simulink model "dab_openloop_fixed_step_interpolation"  (R2024b)
settings: Solver=ode1be  StartTime=0.0  StopTime=T_stop  FixedStep=TFIX  MaxStep=Tsolver  RelTol=1e-05
values from neighbouring files (symbols this model uses):
  Ci = 30e-6*s_f    (= 7.5e-05)    [init.m]
  Co = 44e-6*s_f    (= 0.00011)    [init.m]
  D1_OL = 0.985714    [init.m]
  D2_OL = 1    [init.m]
  D3_OL = 0.045188    [init.m]
  ESR_Ci = 2e-3    (= 0.002)    [init.m]
  ESR_Co = 2e-3    (= 0.002)    [init.m]
  f_sw = 20e3    (= 20000)    [init.m]
  Li = 10e-6*s_f    (= 2.5e-05)    [init.m]
  Lo = 10e-6*s_f    (= 2.5e-05)    [init.m]
  Rd_diode = 8e-3    (= 0.008)    [init.m]
  Ri = 100e-3    (= 0.1)    [init.m]
  Ro = 100e-3    (= 0.1)    [init.m]
  Ron = 3.5e-3    (= 0.0035)    [init.m]
  Rs_snub = 1e5    (= 100000)    [init.m]
  tdead = 200e-9    (= 2e-07)    [init.m]
  TFIX = 20e-9    (= 2e-08)    [init.m]    (also in run_fixed_step_100ns.m = 1e-07; run_fixed_step_20ns.m; run_fixed_step_interpolation_100ns.m = 1e-07; run_fixed_step_interpolation_20ns.m)
  Tp = 1/f_sw    (= 5e-05)    [init.m]
  TR_fn = f_sw    (= 20000)    [init.m]
  TR_Lm = 1    [init.m]
  TR_Pn = 30e3    (= 30000)    [init.m]
  TR_Rm = 1e6    (= 1000000)    [init.m]
  V_cap_init = Vi - Ri*IL0_i    (= 797.500025)    [init.m]
  V_out_init = Vo + Ro*I_OP    (= 454.4444)    [init.m]
  Vf_diode = 3.0    (= 3)    [init.m]
  Vi = 800    [init.m]
  Vo = V_BAT    (= 450)    [init.m]
libraries: spsSeriesRLCBranchLib x16, spsControlledVoltageSourceLib x6, spsCurrentMeasurementLib x3, spsControlledCurrentSourceLib x2, spsGroundLib x2, spsVoltageMeasurementLib x2, spsLinearTransformerLib x1, sps_lib x1
settings Model: Creator=amina  LastModifiedBy=amina
settings SolverCC: MaxConsecutiveMinStep=100
settings DataIOCC: SaveOutput=off  SignalLogging=off  DSMLogging=off  SaveTime=off  ReturnWorkspaceOutputsName=out_analytic

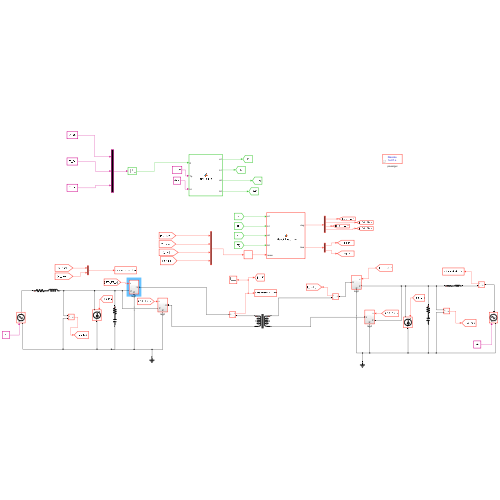
[thumbnail: Simulink's stored preview of the top-level diagram]
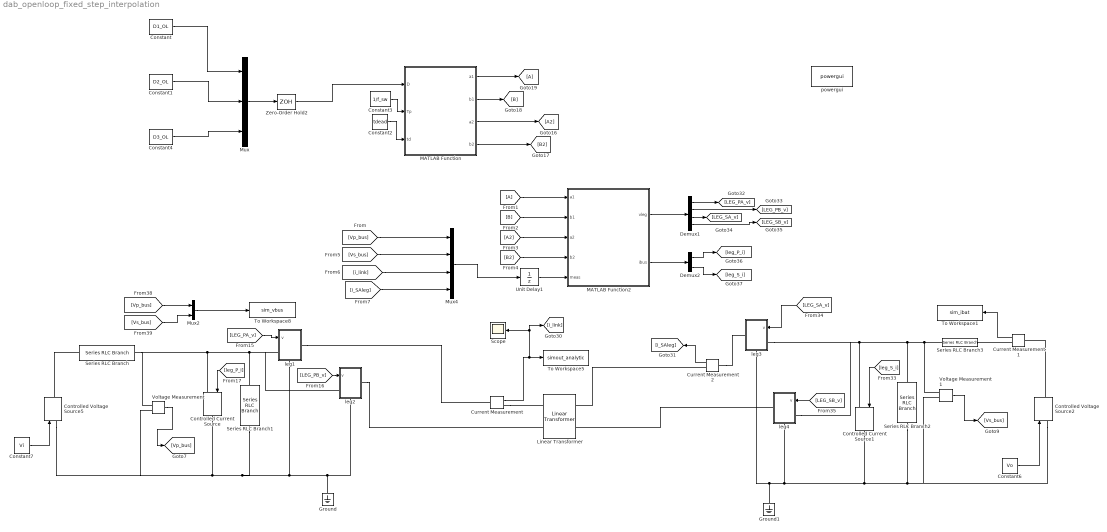
== system dab_openloop_fixed_step_interpolation ==
  Constant : Constant  Value=D1_OL
  Constant1 : Constant  Value=D2_OL
  Constant2 : Constant  Value=tdead
  Constant3 : Constant  Value=1/f_sw
  Constant4 : Constant  Value=D3_OL
  Constant6 : Constant  Value=Vo
  Constant7 : Constant  Value=Vi
  Controlled Current Source : spsControlledCurrentSourceLib/Controlled Current Source  Initialize=off  Source_Type=AC  Amplitude=0  Phase=0  Frequency=0  Measurements=None
  Controlled Current Source1 : spsControlledCurrentSourceLib/Controlled Current Source  Initialize=off  Source_Type=AC  Amplitude=0  Phase=0  Frequency=0  Measurements=None
  Controlled Voltage Source2 : spsControlledVoltageSourceLib/Controlled Voltage Source  Initialize=on  Source_Type=DC  Amplitude=Vo  Phase=0  Frequency=0  Measurements=None
  Controlled Voltage Source5 : spsControlledVoltageSourceLib/Controlled Voltage Source  Initialize=on  Source_Type=DC  Amplitude=Vi  Phase=0  Frequency=0  Measurements=None
  Current Measurement : spsCurrentMeasurementLib/Current Measurement  PhasorSimulation=off  OutputType=Complex  PSBequivalent=0
  Current Measurement1 : spsCurrentMeasurementLib/Current Measurement  PhasorSimulation=off  OutputType=Complex  PSBequivalent=0
  Current Measurement2 : spsCurrentMeasurementLib/Current Measurement  PhasorSimulation=off  OutputType=Complex  PSBequivalent=0
  Demux1 : Demux
  Demux2 : Demux  Outputs=2
  From1 : From
  Goto19 : Goto
  Ground : spsGroundLib/Ground  LConnTagsString=a
  Ground1 : spsGroundLib/Ground  LConnTagsString=a
  Linear Transformer : spsLinearTransformerLib/Linear Transformer  UNITS=SI  NominalPower=[TR_Pn TR_fn]  winding1=TR_W1  winding2=TR_W2  ThreeWindings=off  winding3=[3.15e+05 0.7938 0.084225]  RmLm=[TR_Rm TR_Lm]  Measurements=None  DataType=on
  MATLAB Function : MATLAB Function  TreatAsAtomicUnit=on
  MATLAB Function2 : MATLAB Function  TreatAsAtomicUnit=on
  Mux : Mux  Inputs=3
  Mux2 : Mux  Inputs=2
  Mux4 : Mux
  Scope : Scope
  Series RLC Branch : spsSeriesRLCBranchLib/Series RLC Branch  LConnTagsString=__new0  RConnTagsString=__new0  BranchType=RL  Resistance=Ri  Inductance=Li  SetiL0=on  InitialCurrent=IL0_i  Capacitance=1e-6  Setx0=off  InitialVoltage=0  Measurements=None
  Series RLC Branch1 : spsSeriesRLCBranchLib/Series RLC Branch  LConnTagsString=__new0  RConnTagsString=__new0  BranchType=RC  Resistance=ESR_Ci  Inductance=1e-3  SetiL0=off  InitialCurrent=0  Capacitance=Ci  Setx0=on  InitialVoltage=V_cap_init  Measurements=None
  Series RLC Branch2 : spsSeriesRLCBranchLib/Series RLC Branch  LConnTagsString=__new0  RConnTagsString=__new0  BranchType=RC  Resistance=ESR_Co  Inductance=1e-3  SetiL0=off  InitialCurrent=0  Capacitance=Co  Setx0=on  InitialVoltage=V_out_init  Measurements=None
  Series RLC Branch3 : spsSeriesRLCBranchLib/Series RLC Branch  LConnTagsString=__new0  RConnTagsString=__new0  BranchType=RL  Resistance=Ro  Inductance=Lo  SetiL0=on  InitialCurrent=IL0_o  Capacitance=1e-6  Setx0=off  InitialVoltage=0  Measurements=None
  To Workspace1 : ToWorkspace  VariableName=sim_ibat  SaveFormat=Timeseries  SampleTime=-1
  To Workspace5 : ToWorkspace  VariableName=simout_analytic  SaveFormat=Timeseries  SampleTime=-1
  To Workspace8 : ToWorkspace  VariableName=sim_vbus  SaveFormat=Timeseries  SampleTime=-1
  Unit Delay1 : UnitDelay  InitialCondition=[V_cap_init; V_out_init; 0; 0]  SampleTime=TFIX  HasFrameUpgradeWarning=on
  Voltage Measurement : spsVoltageMeasurementLib/Voltage Measurement  PhasorSimulation=off  OutputType=Complex  PSBequivalent=0
  Voltage Measurement1 : spsVoltageMeasurementLib/Voltage Measurement  PhasorSimulation=off  OutputType=Complex  PSBequivalent=0
  Zero-Order Hold2 : ZeroOrderHold  SampleTime=1/f_sw
  leg1 : Subsystem
      settings: PortSchema="{\"entries\":[{\"content\":{\"sides\":[{\"content\":{\"connectorIds\":[\"In1\",\"LConn1\"]},\"type\":\"ConnectorPlacement.EquallySpacedRectSide\",\"uuid\":\"81142e03-bbe8-4655-b0fc-f40d7cb28308\"},{\"content\":{\"connectorIds\":[\"RConn1\"],\"side\":\"RIGHT\"},\"type\":\"ConnectorPlacement.EquallySpacedRectSide\",\"uuid\":\"8b0fa82a-ef23-4d29-b267-a4b058b7878b\"},{\"content\":{\"side\":\"TOP\"},\"type\":\"ConnectorPlacement.EquallySpacedRectSide\",\"uuid\":\"6ef32b7f-a709-442f-b038-19cc6fffc8df\"},{\"content\":{\"connectorIds\":[\"RConn2\"],\"side\":\"BOTTOM\"},\"type\":\"ConnectorPlacement.EquallySpacedRectSide\",\"uuid\":\"acaab421-7729-4a20-97ce-5be0a5a8c4d3\"}]},\"type\":\"ConnectorPlacement.EquallySpacedConnector\",\"uuid\":\"423ad79b-2f01-454b-b2f3-d9f36115acf4\"}],\"packageUris\":[\"http://schema.mathworks.com/mf0/Connector/R2020b\"],\"version\":\"1.0\"}"
  leg2 : Subsystem
      settings: PortSchema="{\"entries\":[{\"content\":{\"sides\":[{\"content\":{\"connectorIds\":[\"In1\",\"LConn1\"]},\"type\":\"ConnectorPlacement.EquallySpacedRectSide\",\"uuid\":\"81142e03-bbe8-4655-b0fc-f40d7cb28308\"},{\"content\":{\"connectorIds\":[\"RConn1\"],\"side\":\"RIGHT\"},\"type\":\"ConnectorPlacement.EquallySpacedRectSide\",\"uuid\":\"8b0fa82a-ef23-4d29-b267-a4b058b7878b\"},{\"content\":{\"side\":\"TOP\"},\"type\":\"ConnectorPlacement.EquallySpacedRectSide\",\"uuid\":\"6ef32b7f-a709-442f-b038-19cc6fffc8df\"},{\"content\":{\"connectorIds\":[\"RConn2\"],\"side\":\"BOTTOM\"},\"type\":\"ConnectorPlacement.EquallySpacedRectSide\",\"uuid\":\"acaab421-7729-4a20-97ce-5be0a5a8c4d3\"}]},\"type\":\"ConnectorPlacement.EquallySpacedConnector\",\"uuid\":\"423ad79b-2f01-454b-b2f3-d9f36115acf4\"}],\"packageUris\":[\"http://schema.mathworks.com/mf0/Connector/R2020b\"],\"version\":\"1.0\"}"
  leg3 : Subsystem
      settings: PortSchema="{\"entries\":[{\"content\":{\"sides\":[{\"content\":{\"connectorIds\":[\"In1\",\"LConn1\"]},\"type\":\"ConnectorPlacement.EquallySpacedRectSide\",\"uuid\":\"81142e03-bbe8-4655-b0fc-f40d7cb28308\"},{\"content\":{\"connectorIds\":[\"RConn1\"],\"side\":\"RIGHT\"},\"type\":\"ConnectorPlacement.EquallySpacedRectSide\",\"uuid\":\"8b0fa82a-ef23-4d29-b267-a4b058b7878b\"},{\"content\":{\"side\":\"TOP\"},\"type\":\"ConnectorPlacement.EquallySpacedRectSide\",\"uuid\":\"6ef32b7f-a709-442f-b038-19cc6fffc8df\"},{\"content\":{\"connectorIds\":[\"RConn2\"],\"side\":\"BOTTOM\"},\"type\":\"ConnectorPlacement.EquallySpacedRectSide\",\"uuid\":\"acaab421-7729-4a20-97ce-5be0a5a8c4d3\"}]},\"type\":\"ConnectorPlacement.EquallySpacedConnector\",\"uuid\":\"423ad79b-2f01-454b-b2f3-d9f36115acf4\"}],\"packageUris\":[\"http://schema.mathworks.com/mf0/Connector/R2020b\"],\"version\":\"1.0\"}"
  leg4 : Subsystem
      settings: PortSchema="{\"entries\":[{\"content\":{\"sides\":[{\"content\":{\"connectorIds\":[\"In1\",\"LConn1\"]},\"type\":\"ConnectorPlacement.EquallySpacedRectSide\",\"uuid\":\"81142e03-bbe8-4655-b0fc-f40d7cb28308\"},{\"content\":{\"connectorIds\":[\"RConn1\"],\"side\":\"RIGHT\"},\"type\":\"ConnectorPlacement.EquallySpacedRectSide\",\"uuid\":\"8b0fa82a-ef23-4d29-b267-a4b058b7878b\"},{\"content\":{\"side\":\"TOP\"},\"type\":\"ConnectorPlacement.EquallySpacedRectSide\",\"uuid\":\"6ef32b7f-a709-442f-b038-19cc6fffc8df\"},{\"content\":{\"connectorIds\":[\"RConn2\"],\"side\":\"BOTTOM\"},\"type\":\"ConnectorPlacement.EquallySpacedRectSide\",\"uuid\":\"acaab421-7729-4a20-97ce-5be0a5a8c4d3\"}]},\"type\":\"ConnectorPlacement.EquallySpacedConnector\",\"uuid\":\"423ad79b-2f01-454b-b2f3-d9f36115acf4\"}],\"packageUris\":[\"http://schema.mathworks.com/mf0/Connector/R2020b\"],\"version\":\"1.0\"}"
  powergui : sps_lib/powergui  Priority=1  SimulationMode=Discrete  SampleTime=TFIX  frequency=60  Iterations=50  frequencyindice=0  Pbase=100e6  ErrMax=1e-4  UnitsV=kV  UnitsW=MW  buscounter=0  FunctionMessages=off  echomessages=off  EnableUseOfTLC=off  CurrentSourceSwitches=off  DisableSnubberDevices=off  DisableRonSwitches=off  DisableVfSwitches=off  DisplayEquations=off  AutomaticDiscreteSolvers=off  SolverType=Tustin  Interpol=off  ExternalGateDelay=off  methode=off  Ts=100  x0status=blocks  SPID=on  SwTol=0  HookPort=off  NonlinearTolerance=1e-4  nMaxIteration=100  ContinueOnMaxIteration=off  RestoreLinks=warning  ResistiveCurrentMeasurement=off  Frange=[0:2:500]  Ylog=off  Xlog=on  ShowGrid=off  save=off  variable=ZData  structure=0  ZoomFFT=off  StartTime=0.0  cycles=1  DisplayStyle=1  fundamental=60  FreqAxis=off  MaxFrequency=1000  frequencyindicesteady=1  RmsSteady=1  display=off
  wires:
  Constant6/1 -> Controlled Voltage Source2/1
  Constant7/1 -> Controlled Voltage Source5/1
  Current Measurement/1 -> Scope/1, [i_link], To Workspace5/1
  Voltage Measurement/1 -> [Vp_bus]
  Voltage Measurement1/1 -> [Vs_bus]
  [Vs_bus] -> Mux2/2
  Mux2/1 -> To Workspace8/1
  [Vp_bus] -> Mux2/1
  From1/1 -> MATLAB Function2/1(a1)
  [B] -> MATLAB Function2/2(b1)
  [A2] -> MATLAB Function2/3(a2)
  [B2] -> MATLAB Function2/4(b2)
  Current Measurement2/1 -> [i_SAleg]
  [Vp_bus] -> Mux4/1
  [Vs_bus] -> Mux4/2
  [i_link] -> Mux4/3
  [i_SAleg] -> Mux4/4
  Mux4/1 -> Unit Delay1/1
  Unit Delay1/1 -> MATLAB Function2/5(meas)
  MATLAB Function2/2(ibus) -> Demux2/1
  MATLAB Function2/1(vleg) -> Demux1/1
  Demux1/1 -> [LEG_PA_v]
  Demux1/3 -> [LEG_SA_v]
  Demux1/2 -> [LEG_PB_v]
  Demux1/4 -> [LEG_SB_v]
  Demux2/1 -> [leg_P_i]
  Demux2/2 -> [leg_S_i]
  [LEG_PA_v] -> leg1/1(v)
  [LEG_PB_v] -> leg2/1(v)
  [leg_P_i] -> Controlled Current Source/1
  [leg_S_i] -> Controlled Current Source1/1
  [LEG_SA_v] -> leg3/1(v)
  [LEG_SB_v] -> leg4/1(v)
  Mux/1 -> Zero-Order Hold2/1
  Constant/1 -> Mux/1
  Constant1/1 -> Mux/2
  Constant3/1 -> MATLAB Function/2(Tp)
  MATLAB Function/4(b2) -> [B2]
  MATLAB Function/3(a2) -> [A2]
  MATLAB Function/1(a1) -> Goto19/1
  MATLAB Function/2(b1) -> [B]
  Constant2/1 -> MATLAB Function/3(td)
  Constant4/1 -> Mux/3
  Zero-Order Hold2/1 -> MATLAB Function/1(D)
  Current Measurement1/1 -> To Workspace1/1
  connections:
  leg1/RConn1 -- Current Measurement/LConn1
  Voltage Measurement/LConn1 -- Series RLC Branch/RConn1 -- Controlled Current Source/LConn1 -- leg2/LConn1 -- leg1/LConn1 -- Series RLC Branch1/LConn1
  leg1/RConn2 -- Controlled Current Source/RConn1 -- Voltage Measurement/LConn2 -- Controlled Voltage Source5/LConn1 -- Series RLC Branch1/RConn1 -- leg2/RConn2 -- Ground/LConn1
  leg2/RConn1 -- Linear Transformer/LConn2
  Voltage Measurement1/LConn1 -- leg3/LConn1 -- leg4/LConn1 -- Controlled Current Source1/LConn1 -- Series RLC Branch2/LConn1 -- Series RLC Branch3/LConn1
  Voltage Measurement1/LConn2 -- Controlled Voltage Source2/LConn1 -- Series RLC Branch2/RConn1 -- Controlled Current Source1/RConn1 -- leg4/RConn2 -- leg3/RConn2 -- Ground1/LConn1
  leg4/RConn1 -- Linear Transformer/RConn2
  Current Measurement2/RConn1 -- Linear Transformer/RConn1
  Current Measurement/RConn1 -- Linear Transformer/LConn1
  Current Measurement1/RConn1 -- Series RLC Branch3/RConn1
  Controlled Voltage Source2/RConn1 -- Current Measurement1/LConn1
  Controlled Voltage Source5/RConn1 -- Series RLC Branch/LConn1
  Current Measurement2/LConn1 -- leg3/RConn1

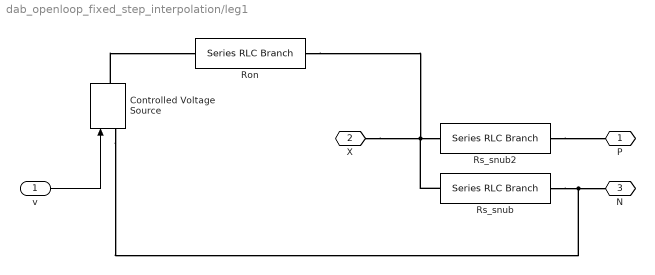
== system dab_openloop_fixed_step_interpolation/leg1 ==
  v : Inport
  Controlled Voltage Source : spsControlledVoltageSourceLib/Controlled Voltage Source  Initialize=off  Source_Type=AC  Amplitude=0  Phase=0  Frequency=0  Measurements=None
  Ron : spsSeriesRLCBranchLib/Series RLC Branch  LConnTagsString=__new0  RConnTagsString=__new0  BranchType=R  Resistance=Ron  Inductance=Li  SetiL0=on  InitialCurrent=IL0_i  Capacitance=1e-6  Setx0=off  InitialVoltage=0  Measurements=None
  Rs_snub : spsSeriesRLCBranchLib/Series RLC Branch  LConnTagsString=__new0  RConnTagsString=__new0  BranchType=R  Resistance=Rs_snub  Inductance=Li  SetiL0=on  InitialCurrent=IL0_i  Capacitance=1e-6  Setx0=off  InitialVoltage=0  Measurements=None
  Rs_snub2 : spsSeriesRLCBranchLib/Series RLC Branch  LConnTagsString=__new0  RConnTagsString=__new0  BranchType=R  Resistance=Rs_snub  Inductance=Li  SetiL0=on  InitialCurrent=IL0_i  Capacitance=1e-6  Setx0=off  InitialVoltage=0  Measurements=None
  " P" : PMIOPort  Side=Left
  X : PMIOPort  Port=2  Side=Right
  N : PMIOPort  Port=3  Side=Right
  wires:
  v/1 -> Controlled Voltage Source/1
  connections:
  Rs_snub2/RConn1 -- " P"/RConn1
  Rs_snub/LConn1 -- Rs_snub2/LConn1 -- X/RConn1 -- Ron/RConn1
  Controlled Voltage Source/LConn1 -- Rs_snub/RConn1 -- N/RConn1
  Controlled Voltage Source/RConn1 -- Ron/LConn1

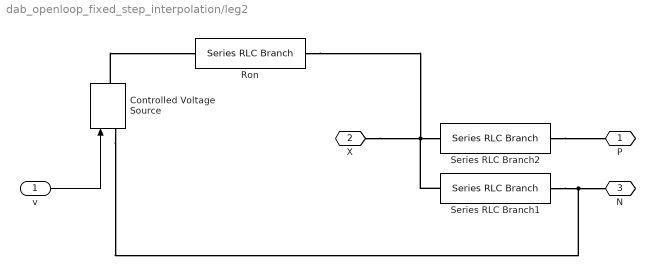
== system dab_openloop_fixed_step_interpolation/leg2 ==
  v : Inport
  Controlled Voltage Source : spsControlledVoltageSourceLib/Controlled Voltage Source  Initialize=off  Source_Type=AC  Amplitude=0  Phase=0  Frequency=0  Measurements=None
  Ron : spsSeriesRLCBranchLib/Series RLC Branch  LConnTagsString=__new0  RConnTagsString=__new0  BranchType=R  Resistance=Ron  Inductance=Li  SetiL0=on  InitialCurrent=IL0_i  Capacitance=1e-6  Setx0=off  InitialVoltage=0  Measurements=None
  Series RLC Branch1 : spsSeriesRLCBranchLib/Series RLC Branch  LConnTagsString=__new0  RConnTagsString=__new0  BranchType=R  Resistance=Rs_snub  Inductance=Li  SetiL0=on  InitialCurrent=IL0_i  Capacitance=1e-6  Setx0=off  InitialVoltage=0  Measurements=None
  Series RLC Branch2 : spsSeriesRLCBranchLib/Series RLC Branch  LConnTagsString=__new0  RConnTagsString=__new0  BranchType=R  Resistance=Rs_snub  Inductance=Li  SetiL0=on  InitialCurrent=IL0_i  Capacitance=1e-6  Setx0=off  InitialVoltage=0  Measurements=None
  " P" : PMIOPort  Side=Left
  X : PMIOPort  Port=2  Side=Right
  N : PMIOPort  Port=3  Side=Right
  wires:
  v/1 -> Controlled Voltage Source/1
  connections:
  Series RLC Branch2/RConn1 -- " P"/RConn1
  Series RLC Branch1/LConn1 -- Series RLC Branch2/LConn1 -- X/RConn1 -- Ron/RConn1
  Controlled Voltage Source/LConn1 -- Series RLC Branch1/RConn1 -- N/RConn1
  Controlled Voltage Source/RConn1 -- Ron/LConn1

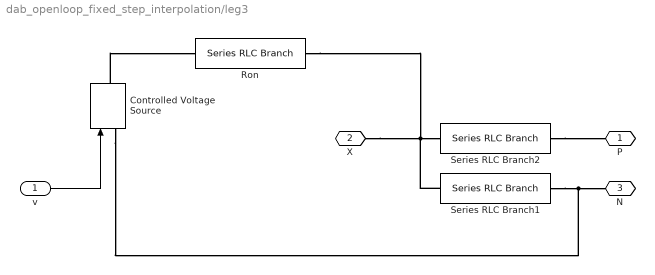
== system dab_openloop_fixed_step_interpolation/leg3 ==
  v : Inport
  Controlled Voltage Source : spsControlledVoltageSourceLib/Controlled Voltage Source  Initialize=off  Source_Type=AC  Amplitude=0  Phase=0  Frequency=0  Measurements=None
  Ron : spsSeriesRLCBranchLib/Series RLC Branch  LConnTagsString=__new0  RConnTagsString=__new0  BranchType=R  Resistance=Ron  Inductance=Li  SetiL0=on  InitialCurrent=IL0_i  Capacitance=1e-6  Setx0=off  InitialVoltage=0  Measurements=None
  Series RLC Branch1 : spsSeriesRLCBranchLib/Series RLC Branch  LConnTagsString=__new0  RConnTagsString=__new0  BranchType=R  Resistance=Rs_snub  Inductance=Li  SetiL0=on  InitialCurrent=IL0_i  Capacitance=1e-6  Setx0=off  InitialVoltage=0  Measurements=None
  Series RLC Branch2 : spsSeriesRLCBranchLib/Series RLC Branch  LConnTagsString=__new0  RConnTagsString=__new0  BranchType=R  Resistance=Rs_snub  Inductance=Li  SetiL0=on  InitialCurrent=IL0_i  Capacitance=1e-6  Setx0=off  InitialVoltage=0  Measurements=None
  " P" : PMIOPort  Side=Left
  X : PMIOPort  Port=2  Side=Right
  N : PMIOPort  Port=3  Side=Right
  wires:
  v/1 -> Controlled Voltage Source/1
  connections:
  Series RLC Branch2/RConn1 -- " P"/RConn1
  Series RLC Branch1/LConn1 -- Series RLC Branch2/LConn1 -- X/RConn1 -- Ron/RConn1
  Controlled Voltage Source/LConn1 -- Series RLC Branch1/RConn1 -- N/RConn1
  Controlled Voltage Source/RConn1 -- Ron/LConn1

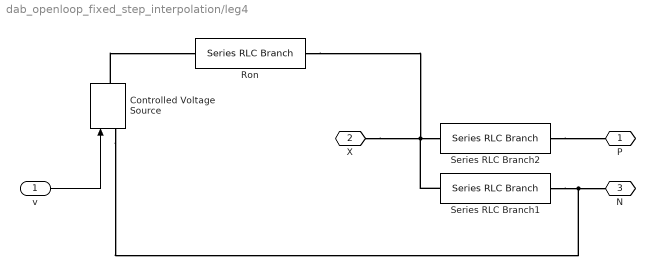
== system dab_openloop_fixed_step_interpolation/leg4 ==
  v : Inport
  Controlled Voltage Source : spsControlledVoltageSourceLib/Controlled Voltage Source  Initialize=off  Source_Type=AC  Amplitude=0  Phase=0  Frequency=0  Measurements=None
  Ron : spsSeriesRLCBranchLib/Series RLC Branch  LConnTagsString=__new0  RConnTagsString=__new0  BranchType=R  Resistance=Ron  Inductance=Li  SetiL0=on  InitialCurrent=IL0_i  Capacitance=1e-6  Setx0=off  InitialVoltage=0  Measurements=None
  Series RLC Branch1 : spsSeriesRLCBranchLib/Series RLC Branch  LConnTagsString=__new0  RConnTagsString=__new0  BranchType=R  Resistance=Rs_snub  Inductance=Li  SetiL0=on  InitialCurrent=IL0_i  Capacitance=1e-6  Setx0=off  InitialVoltage=0  Measurements=None
  Series RLC Branch2 : spsSeriesRLCBranchLib/Series RLC Branch  LConnTagsString=__new0  RConnTagsString=__new0  BranchType=R  Resistance=Rs_snub  Inductance=Li  SetiL0=on  InitialCurrent=IL0_i  Capacitance=1e-6  Setx0=off  InitialVoltage=0  Measurements=None
  " P" : PMIOPort  Side=Left
  X : PMIOPort  Port=2  Side=Right
  N : PMIOPort  Port=3  Side=Right
  wires:
  v/1 -> Controlled Voltage Source/1
  connections:
  Series RLC Branch2/RConn1 -- " P"/RConn1
  Series RLC Branch1/LConn1 -- Series RLC Branch2/LConn1 -- X/RConn1 -- Ron/RConn1
  Controlled Voltage Source/LConn1 -- Series RLC Branch1/RConn1 -- N/RConn1
  Controlled Voltage Source/RConn1 -- Ron/LConn1

== matlab function dab_openloop_fixed_step_interpolation/MATLAB Function ==
  settings: updateMethod=DISCRETE  sampleTime=1/f_sw
  data: D input; a1 output size=[8 1]; Tp input; td input; b1 output size=[8 1]; a2 output size=[8 1]; b2 output size=[8 1]
function [a1, b1, a2, b2] = gate_block(D, Tp, td)
    persistent s0 p
    if isempty(s0)
        cu = [0; D(1); D(3); D(3) + D(2)];
        u  = mod(cu*Tp/2, Tp);   d = mod((cu + 1)*Tp/2, Tp);
        s0 = u > d;   p = max(u, d) - Tp;
    end
    [a1, b1, a2, b2, s0, p] = gate_core(D, Tp, td, s0, p);
end

== matlab function dab_openloop_fixed_step_interpolation/MATLAB Function2 ==
  settings: updateMethod=DISCRETE  sampleTime=TFIX
  data: a1 input; vleg output size=4; b1 input; a2 input; b2 input; meas input; ibus output size=2; Tp parameter; TFIX parameter; Rd_diode parameter; Vf_diode parameter; Ron parameter
function [vleg, ibus] = bridge_interp_block(a1, b1, a2, b2, meas, Tp, TFIX, Rd_diode, Vf_diode, Ron)
persistent j
if isempty(j), j = 0; end
NP = round(Tp/TFIX);
k  = mod(j, NP);
t0 = k*TFIX;   t1 = t0 + TFIX;
A  = [a1(:), b1(:), a2(:), b2(:)];

f = zeros(8, 1);
for s = 1:8
    f(s) = (max(0, min(A(s,2), t1) - max(A(s,1), t0)) + max(0, min(A(s,4), t1) - max(A(s,3), t0))) / TFIX;
end

Vp = meas(1);   Vs = meas(2);   ip = meas(3);   is = meas(4);
il = [ip; -ip; is; -is];
Vb = [Vp; Vp; Vs; Vs];
vleg = zeros(4, 1);   hi = zeros(4, 1);
for leg = 1:4
    fh = f(2*leg-1);   fl = f(2*leg);
    fd = max(0, 1 - fh - fl);
    if il(leg) < 0
        hi(leg) = fh + fd;   sd = 1;
    else
        hi(leg) = fh;        sd = -1;
    end
    vleg(leg) = hi(leg)*Vb(leg) + fd*(sd*Vf_diode - (Rd_diode - Ron)*il(leg));
end
ibus = [hi(1)*il(1) + hi(2)*il(2);  hi(3)*il(3) + hi(4)*il(4)];
j = j + 1;
end
